simulink library "lib_SecCtrl_PilotNodes"  (R2026a)
settings: Solver=VariableStepAuto
undefined symbols (not defined in the file): buses_lf, fref
settings Model: Creator=atomas  LastModifiedBy=atomas

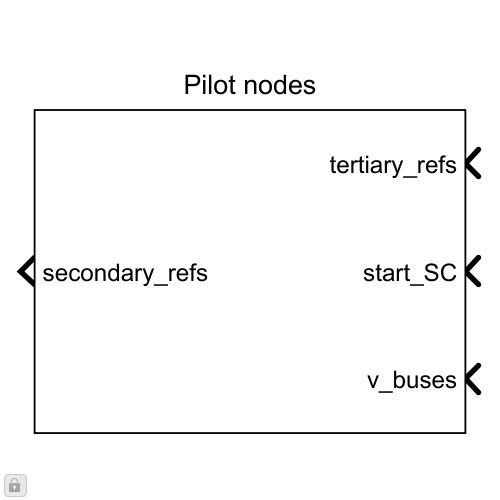
[thumbnail: Simulink's stored preview of the top-level diagram]
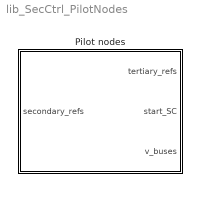
== system lib_SecCtrl_PilotNodes ==
  Pilot nodes : Subsystem  VariantControl=Pilot nodes

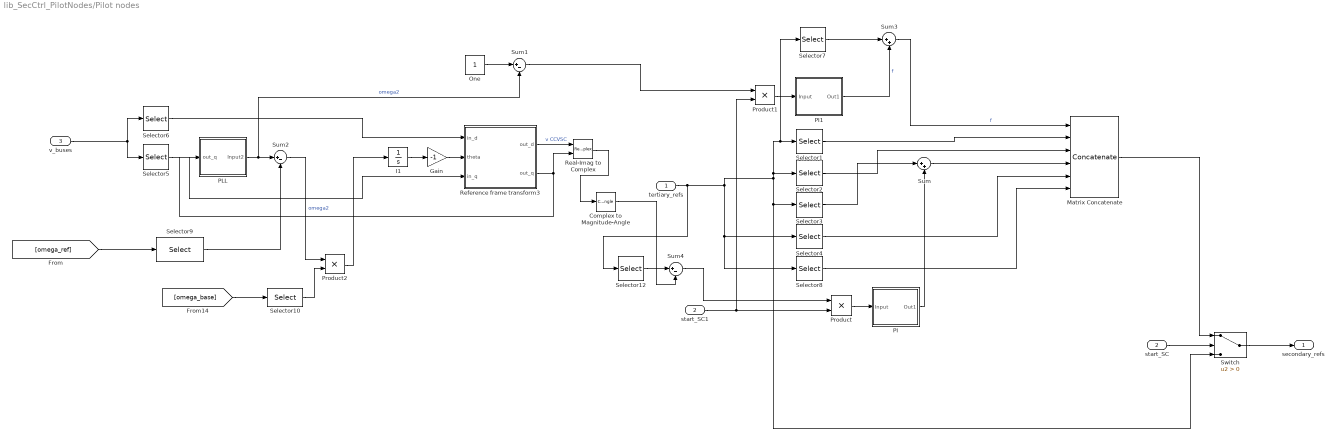
== system lib_SecCtrl_PilotNodes/Pilot nodes ==
  tertiary_refs : Inport
  start_SC : Inport  Port=2
  v_buses : Inport  Port=3
  Complex to Magnitude-Angle : ComplexToMagnitudeAngle  Output=Magnitude
  Gain : Gain  Gain=-1
  I1 : Integrator
  Matrix Concatenate : Concatenate  NumInputs=6  Mode=Multidimensional array
  One : Constant  OutDataTypeStr=Inherit: Inherit via back propagation
  PI : Subsystem
  PI1 : Subsystem
  PLL : Subsystem
  Product : Product
  Product1 : Product
  Product2 : Product
  Real-Imag to Complex : RealImagToComplex
  Reference frame transform3 : Subsystem
  Selector1 : Selector  NumberOfDimensions=2  InputPortWidth=3  IndexOptions=Index vector (dialog),Select all  Indices=2,1  OutputSizes=1,1
  Selector10 : Selector  InputPortWidth=length(fref.ref_units)  IndexOptions=Index vector (dialog)  Indices=fref.Fb_units  OutputSizes=1
  Selector12 : Selector  NumberOfDimensions=2  InputPortWidth=3  IndexOptions=Index vector (dialog),Select all  Indices=3,1  OutputSizes=1,1
  Selector2 : Selector  NumberOfDimensions=2  InputPortWidth=3  IndexOptions=Index vector (dialog),Select all  Indices=3,1  OutputSizes=1,1
  Selector3 : Selector  NumberOfDimensions=2  InputPortWidth=3  IndexOptions=Index vector (dialog),Select all  Indices=4,1  OutputSizes=1,1
  Selector4 : Selector  NumberOfDimensions=2  InputPortWidth=3  IndexOptions=Index vector (dialog),Select all  Indices=5,1  OutputSizes=1,1
  Selector5 : Selector  NumberOfDimensions=2  InputPortWidth=3  IndexOptions=Index vector (dialog),Index vector (dialog)  Indices=2,buses_lf  OutputSizes=1,1
  Selector6 : Selector  NumberOfDimensions=2  InputPortWidth=3  IndexOptions=Index vector (dialog),Index vector (dialog)  Indices=1,buses_lf  OutputSizes=1,1
  Selector7 : Selector  NumberOfDimensions=2  InputPortWidth=3  IndexOptions=Index vector (dialog),Select all  Indices=1,1  OutputSizes=1,1
  Selector8 : Selector  NumberOfDimensions=2  InputPortWidth=3  IndexOptions=Index vector (dialog),Select all  Indices=6,1  OutputSizes=1,1
  Selector9 : Selector  InputPortWidth=length(fref.ref_units)  IndexOptions=Index vector (dialog)  Indices=fref.Fb_units  OutputSizes=1
  Sum : Sum  Inputs=|++
  Sum1 : Sum  Inputs=|+-
  Sum2 : Sum  Inputs=|+-
  Sum3 : Sum  Inputs=|++
  Sum4 : Sum  Inputs=|+-
  Switch : Switch  Criteria=u2 > Threshold  SaturateOnIntegerOverflow=off  InputSameDT=off
  start_SC1 : InportShadow  Port=2
  secondary_refs : Outport
  wires:
  Sum4/1 -> Product/1
  Real-Imag to Complex/1 -> Complex to Magnitude-Angle/1
  Reference frame transform3/1(out_d) -> Real-Imag to Complex/1  "v CCVSC"
  Complex to Magnitude-Angle/1 -> Sum4/2
  Selector12/1 -> Sum4/1
  PI/1(Out1) -> Sum/2
  [omega_base] -> Selector10/1
  Selector10/1 -> Product2/2
  [omega_ref] -> Selector9/1
  PI1/1(Out1) -> Sum3/2  "f"
  Selector7/1 -> Sum3/1
  Sum1/1 -> Product1/1
  Gain/1 -> Reference frame transform3/2(theta)
  Selector9/1 -> Sum2/2
  PLL/1(Input2) -> Sum2/1, Sum1/2  "omega2"
  One/1 -> Sum1/1
  I1/1 -> Gain/1
  Product2/1 -> I1/1
  Reference frame transform3/2(out_q) -> Real-Imag to Complex/2, PLL/1(out_q)
  Selector6/1 -> Reference frame transform3/1(in_d)
  v_buses/1 -> Selector6/1, Selector5/1
  Selector5/1 -> Reference frame transform3/3(in_q)
  Sum2/1 -> Product2/1  "omega2"
  Product1/1 -> PI1/1(Input)
  start_SC1/1 -> Product1/2, Product/2
  Selector8/1 -> Matrix Concatenate/6
  Sum3/1 -> Matrix Concatenate/1  "f"
  Product/1 -> PI/1(Input)
  tertiary_refs/1 -> Selector4/1, Selector8/1, Selector3/1, Switch/3, Selector2/1, Selector1/1, Selector7/1, Selector12/1
  Switch/1 -> secondary_refs/1
  start_SC/1 -> Switch/2
  Selector4/1 -> Matrix Concatenate/5
  Selector2/1 -> Matrix Concatenate/3
  Selector1/1 -> Matrix Concatenate/2
  Selector3/1 -> Sum/1
  Matrix Concatenate/1 -> Switch/1
  Sum/1 -> Matrix Concatenate/4

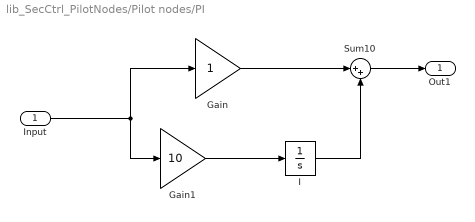
== system lib_SecCtrl_PilotNodes/Pilot nodes/PI ==
  Input : Inport
  Gain : Gain
  Gain1 : Gain  Gain=10
  I : Integrator
  Sum10 : Sum  Inputs=|++
  Out1 : Outport
  wires:
  Gain1/1 -> I/1
  I/1 -> Sum10/2
  Gain/1 -> Sum10/1
  Sum10/1 -> Out1/1
  Input/1 -> Gain/1, Gain1/1

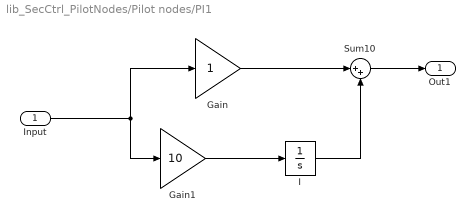
== system lib_SecCtrl_PilotNodes/Pilot nodes/PI1 ==
  Input : Inport
  Gain : Gain
  Gain1 : Gain  Gain=10
  I : Integrator
  Sum10 : Sum  Inputs=|++
  Out1 : Outport
  wires:
  Input/1 -> Gain1/1, Gain/1
  Sum10/1 -> Out1/1
  Gain/1 -> Sum10/1
  I/1 -> Sum10/2
  Gain1/1 -> I/1

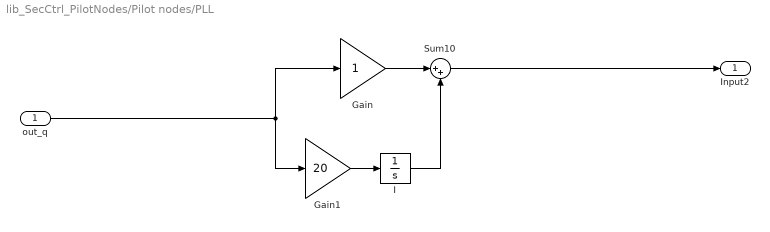
== system lib_SecCtrl_PilotNodes/Pilot nodes/PLL ==
  out_q : Inport
  Gain : Gain
  Gain1 : Gain  Gain=20
  I : Integrator  InitialCondition=1
  Sum10 : Sum  Inputs=|++
  Input2 : Outport
  wires:
  Sum10/1 -> Input2/1
  out_q/1 -> Gain1/1, Gain/1
  Gain1/1 -> I/1
  Gain/1 -> Sum10/1
  I/1 -> Sum10/2

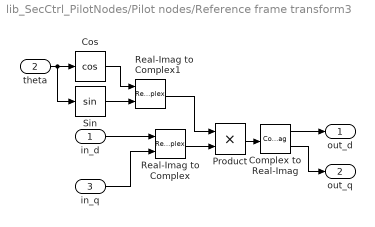
== system lib_SecCtrl_PilotNodes/Pilot nodes/Reference frame transform3 ==
  in_d : Inport
  theta : Inport  Port=2
  in_q : Inport  Port=3
  Complex to Real-Imag : ComplexToRealImag
  Cos : Trigonometry  SCDEnableBlockLinearizationSpecification=on  Operator=cos
  Product : Product
  Real-Imag to Complex : RealImagToComplex
  Real-Imag to Complex1 : RealImagToComplex
  Sin : Trigonometry  SCDEnableBlockLinearizationSpecification=on
  out_d : Outport
  out_q : Outport  Port=2
  wires:
  in_d/1 -> Real-Imag to Complex/1
  in_q/1 -> Real-Imag to Complex/2
  Complex to Real-Imag/1 -> out_d/1
  Sin/1 -> Real-Imag to Complex1/2
  Cos/1 -> Real-Imag to Complex1/1
  theta/1 -> Cos/1, Sin/1
  Product/1 -> Complex to Real-Imag/1
  Real-Imag to Complex/1 -> Product/2
  Real-Imag to Complex1/1 -> Product/1
  Complex to Real-Imag/2 -> out_q/1
